simulink model "firstcircuit"  (R2022b)
settings: Solver=VariableStepAuto  StartTime=0.0  StopTime=0.10  RelTol=1e-3
libraries: ee_lib x9, fl_lib x4, nesl_utility x4
settings Model: Creator=fuad  LastModifiedBy=fuad

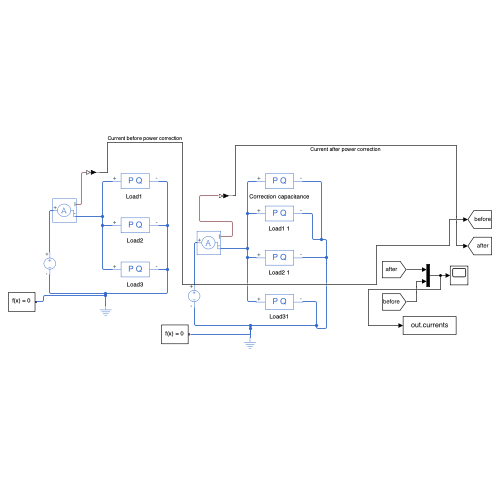
[thumbnail: Simulink's stored preview of the top-level diagram]
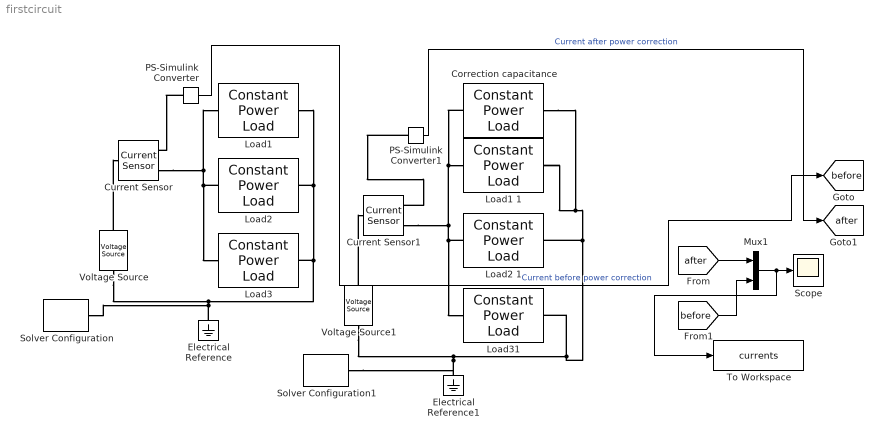
== system firstcircuit ==
  Correction capacitance : ee_lib/Passive/Constant Power Load  load_type=ee.enum.dc_ac.ac  consumed_power=100 W  min_supply_voltage=20 V  G_reverse=1e-6 S  deltaV=1e-3 V  active_power=0.0000000001 W  reactive_power=-5849.34 A*V  f0=50 Hz  Vrms_min=200 V  enable_fault=simscape.enum.onoff.off  fault_action=simscape.enum.assert.action.none  t_fault=1 s  open_conductance=1e-4 S
      settings: InternalSimscapePortConfiguration="{\"Bottom\":[],\"Left\":[{\"id\":\"p\",\"label\":\"+\",\"type\":\"foundation.electrical.electrical\"}],\"Right\":[{\"id\":\"n\",\"label\":\"-\",\"type\":\"foundation.electrical.electrical\"}],\"Top\":[]}"
  Current Sensor : fl_lib/Electrical/Electrical Sensors/Current Sensor
  Current Sensor1 : fl_lib/Electrical/Electrical Sensors/Current Sensor
  Electrical Reference : fl_lib/Electrical/Electrical Elements/Electrical Reference
  Electrical Reference1 : fl_lib/Electrical/Electrical Elements/Electrical Reference
  "Load1 " : ee_lib/Passive/Constant Power Load  load_type=ee.enum.dc_ac.ac  consumed_power=100 W  min_supply_voltage=20 V  G_reverse=1e-6 S  deltaV=1e-3 V  active_power=19042 W  reactive_power=20528 A*V  f0=50 Hz  Vrms_min=200 V  enable_fault=simscape.enum.onoff.off  fault_action=simscape.enum.assert.action.none  t_fault=1 s  open_conductance=1e-4 S
      settings: InternalSimscapePortConfiguration="{\"Bottom\":[],\"Left\":[{\"id\":\"p\",\"label\":\"+\",\"type\":\"foundation.electrical.electrical\"}],\"Right\":[{\"id\":\"n\",\"label\":\"-\",\"type\":\"foundation.electrical.electrical\"}],\"Top\":[]}"
  Load1 1 : ee_lib/Passive/Constant Power Load  load_type=ee.enum.dc_ac.ac  consumed_power=100 W  min_supply_voltage=20 V  G_reverse=1e-6 S  deltaV=1e-3 V  active_power=19042 W  reactive_power=20528 A*V  f0=50 Hz  Vrms_min=200 V  enable_fault=simscape.enum.onoff.off  fault_action=simscape.enum.assert.action.none  t_fault=1 s  open_conductance=1e-4 S
      settings: InternalSimscapePortConfiguration="{\"Bottom\":[],\"Left\":[{\"id\":\"p\",\"label\":\"+\",\"type\":\"foundation.electrical.electrical\"}],\"Right\":[{\"id\":\"n\",\"label\":\"-\",\"type\":\"foundation.electrical.electrical\"}],\"Top\":[]}"
  Load2 : ee_lib/Passive/Constant Power Load  load_type=ee.enum.dc_ac.ac  consumed_power=100 W  min_supply_voltage=20 V  G_reverse=1e-6 S  deltaV=1e-3 V  active_power=5000 W  reactive_power=-3489.6 A*V  f0=50 Hz  Vrms_min=200 V  enable_fault=simscape.enum.onoff.off  fault_action=simscape.enum.assert.action.none  t_fault=1 s  open_conductance=1e-4 S
      settings: InternalSimscapePortConfiguration="{\"Bottom\":[],\"Left\":[{\"id\":\"p\",\"label\":\"+\",\"type\":\"foundation.electrical.electrical\"}],\"Right\":[{\"id\":\"n\",\"label\":\"-\",\"type\":\"foundation.electrical.electrical\"}],\"Top\":[]}"
  Load2 1 : ee_lib/Passive/Constant Power Load  load_type=ee.enum.dc_ac.ac  consumed_power=100 W  min_supply_voltage=20 V  G_reverse=1e-6 S  deltaV=1e-3 V  active_power=5000 W  reactive_power=-3489.6 A*V  f0=50 Hz  Vrms_min=200 V  enable_fault=simscape.enum.onoff.off  fault_action=simscape.enum.assert.action.none  t_fault=1 s  open_conductance=1e-4 S
      settings: InternalSimscapePortConfiguration="{\"Bottom\":[],\"Left\":[{\"id\":\"p\",\"label\":\"+\",\"type\":\"foundation.electrical.electrical\"}],\"Right\":[{\"id\":\"n\",\"label\":\"-\",\"type\":\"foundation.electrical.electrical\"}],\"Top\":[]}"
  Load3 : ee_lib/Passive/Constant Power Load  load_type=ee.enum.dc_ac.ac  consumed_power=100 W  min_supply_voltage=20 V  G_reverse=1e-6 S  deltaV=1e-3 V  active_power=10000 W  reactive_power=0 A*V  f0=50 Hz  Vrms_min=200 V  enable_fault=simscape.enum.onoff.off  fault_action=simscape.enum.assert.action.none  t_fault=1 s  open_conductance=1e-4 S
      settings: InternalSimscapePortConfiguration="{\"Bottom\":[],\"Left\":[{\"id\":\"p\",\"label\":\"+\",\"type\":\"foundation.electrical.electrical\"}],\"Right\":[{\"id\":\"n\",\"label\":\"-\",\"type\":\"foundation.electrical.electrical\"}],\"Top\":[]}"
  Load31 : ee_lib/Passive/Constant Power Load  load_type=ee.enum.dc_ac.ac  consumed_power=100 W  min_supply_voltage=20 V  G_reverse=1e-6 S  deltaV=1e-3 V  active_power=10000 W  reactive_power=0 A*V  f0=50 Hz  Vrms_min=200 V  enable_fault=simscape.enum.onoff.off  fault_action=simscape.enum.assert.action.none  t_fault=1 s  open_conductance=1e-4 S
      settings: InternalSimscapePortConfiguration="{\"Bottom\":[],\"Left\":[{\"id\":\"p\",\"label\":\"+\",\"type\":\"foundation.electrical.electrical\"}],\"Right\":[{\"id\":\"n\",\"label\":\"-\",\"type\":\"foundation.electrical.electrical\"}],\"Top\":[]}"
  Mux1 : Mux  Inputs=2
  PS-Simulink Converter : nesl_utility/PS-Simulink Converter  PhysicalDomain=network_engine_domain  SubClassName=ps_output  LeftPortType=input  RightPortType=output  PseudoPeriodic=off  Frequencies=[]  VectorFormat=inherit  Unit=inherit  AffineConversion=off
  PS-Simulink Converter1 : nesl_utility/PS-Simulink Converter  PhysicalDomain=network_engine_domain  SubClassName=ps_output  LeftPortType=input  RightPortType=output  PseudoPeriodic=off  Frequencies=[]  VectorFormat=inherit  Unit=inherit  AffineConversion=off
  Scope : Scope
  Solver Configuration : nesl_utility/Solver Configuration  PhysicalDomain=network_engine_domain  SubClassName=solver  LeftPortType=input  RightPortType=generic  Tones=[]  Harmonics=[]  SimulateNoise=off  Profile=off  UseLocalSampling=off  EnableSwitchedLinearOptims=on  FrequencyDomain=off  UseCCode=off  RelTol=0.001  AbsTol=0.001  MinStep=1e-09  ToWorkspace=off  RevertToSquareIcSolve=off  NumHomotopyIterations=100  PhasorMode=off  PhasorModeNumHarmonics=1  ConsistencySolver=NEWTON_XTOL_AFTER_FTOL  IndexReductionMethod=DerivativeReplacement  DoDC=off  ResidualTolerance=1e-09  ConsistencyTolSource=GLOBAL  ConsistencyAbsTol=0.001  ConsistencyRelTol=0.001  ConsistencyTolFactor=0.001  UseLocalSolver=off  LocalSolverChoice=NE_BACKWARD_EULER_ADVANCER  ResolveIndetEquations=on  FunctionEvalNumThread=1  LocalSolverSampleTime=0.001  DoFixedCost=off  MaxNonlinIter=3  MaxModeIter=2  ComputeImpulses=off  ImpulseIterations=2  LinearAlgebra=auto  LinearAlgebraNumThread=0  EquationFormulation=NE_TIME_EF  DelaysMemoryBudget=1024  AutomaticFiltering=on  FilteringTimeConstant=0.001  PartitionStorageMethod=AS_NEEDED  PartitionMemoryBudget=1024  PartitionMethod=ROBUST
  Solver Configuration1 : nesl_utility/Solver Configuration  PhysicalDomain=network_engine_domain  SubClassName=solver  LeftPortType=input  RightPortType=generic  Tones=[]  Harmonics=[]  SimulateNoise=off  Profile=off  UseLocalSampling=off  EnableSwitchedLinearOptims=on  FrequencyDomain=off  UseCCode=off  RelTol=0.001  AbsTol=0.001  MinStep=1e-09  ToWorkspace=off  RevertToSquareIcSolve=off  NumHomotopyIterations=100  PhasorMode=off  PhasorModeNumHarmonics=1  ConsistencySolver=NEWTON_XTOL_AFTER_FTOL  IndexReductionMethod=DerivativeReplacement  DoDC=off  ResidualTolerance=1e-09  ConsistencyTolSource=GLOBAL  ConsistencyAbsTol=0.001  ConsistencyRelTol=0.001  ConsistencyTolFactor=0.001  UseLocalSolver=off  LocalSolverChoice=NE_BACKWARD_EULER_ADVANCER  ResolveIndetEquations=on  FunctionEvalNumThread=1  LocalSolverSampleTime=0.001  DoFixedCost=off  MaxNonlinIter=3  MaxModeIter=2  ComputeImpulses=off  ImpulseIterations=2  LinearAlgebra=auto  LinearAlgebraNumThread=0  EquationFormulation=NE_TIME_EF  DelaysMemoryBudget=1024  AutomaticFiltering=on  FilteringTimeConstant=0.001  PartitionStorageMethod=AS_NEEDED  PartitionMemoryBudget=1024  PartitionMethod=ROBUST
  To Workspace : ToWorkspace  VariableName=currents  SampleTime=-1
  Voltage Source : ee_lib/Sources/Voltage Source  dc_voltage=0 V  ac_voltage=230*sqrt(2) V  ac_shift=0 rad  ac_frequency=50 Hz  noise_mode=ee.enum.sources.noise.Disabled  PSD=0 V^2/Hz  sample_time=1e-3 s  repeatability=ee.enum.sources.repeatability.NotRepeatable  user_seed=0  auto_seed=3499211588  i_specify=off  i_priority=None  i=0 A  i_nominal_specify=off  i_nominal_unit=A  i_nominal_value=1  v_specify=off  v_priority=None  v=0 V  v_nominal_specify=off  v_nominal_unit=V  v_nominal_value=1
  Voltage Source1 : ee_lib/Sources/Voltage Source  dc_voltage=0 V  ac_voltage=230*sqrt(2) V  ac_shift=0 rad  ac_frequency=50 Hz  noise_mode=ee.enum.sources.noise.Disabled  PSD=0 V^2/Hz  sample_time=1e-3 s  repeatability=ee.enum.sources.repeatability.NotRepeatable  user_seed=0  auto_seed=3890346746  i_specify=off  i_priority=None  i=0 A  i_nominal_specify=off  i_nominal_unit=A  i_nominal_value=1  v_specify=off  v_priority=None  v=0 V  v_nominal_specify=off  v_nominal_unit=V  v_nominal_value=1
  tag scope: after=global, before=global
  wires:
  PS-Simulink Converter/1 -> [before]  "Current before power correction"
  PS-Simulink Converter1/1 -> [after]  "Current after power correction"
  Mux1/1 -> Scope/1, To Workspace/1
  [after] -> Mux1/1
  [before] -> Mux1/2
  connections:
  Load2/LConn1 -- Load3/LConn1 -- "Load1 "/LConn1 -- Current Sensor/RConn2
  "Load1 "/RConn1 -- Solver Configuration/RConn1 -- Electrical Reference/LConn1 -- Voltage Source/RConn1 -- Load3/RConn1 -- Load2/RConn1
  Voltage Source/LConn1 -- Current Sensor/LConn1
  PS-Simulink Converter/LConn1 -- Current Sensor/RConn1
  Current Sensor1/RConn2 -- Load2 1/LConn1 -- Load31/LConn1 -- Correction capacitance/LConn1 -- Load1 1/LConn1
  Voltage Source1/RConn1 -- Solver Configuration1/RConn1 -- Electrical Reference1/LConn1 -- Load1 1/RConn1 -- Correction capacitance/RConn1 -- Load2 1/RConn1 -- Load31/RConn1
  Voltage Source1/LConn1 -- Current Sensor1/LConn1
  PS-Simulink Converter1/LConn1 -- Current Sensor1/RConn1
